simulink model "GaN_Cauer_Figure14"  (R2022b)
settings: Solver=ode15s  StartTime=-5e-6  StopTime=45e-6  MaxStep=2e-9  RelTol=1e-9  AbsTol=1e-10
model workspace (MAT data in the model file):
  C = [8e-05 0.00074 0.0065 0.002]
  R = [0.015 0.23 0.24 0.015]
settings Model: Creator=Greatlovers  LastModifiedBy=Greatlovers

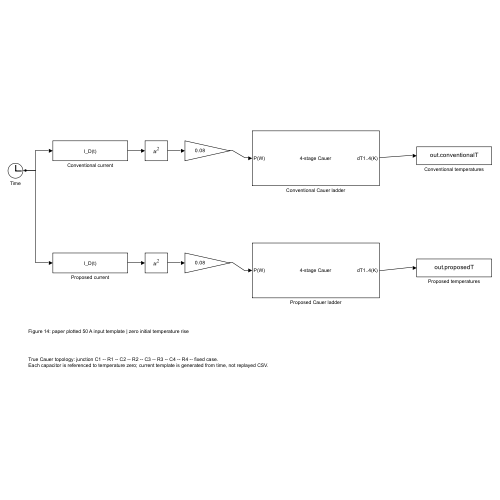
[thumbnail: Simulink's stored preview of the top-level diagram]
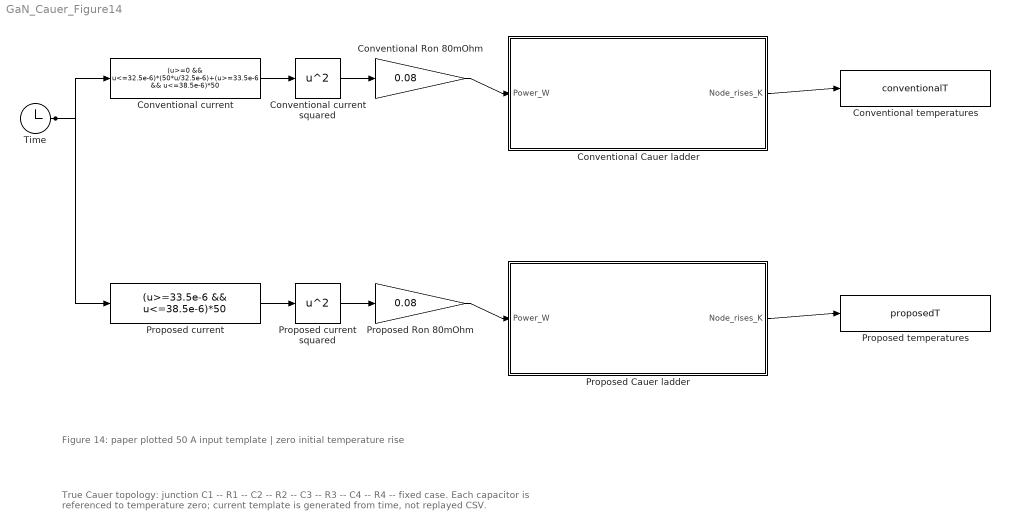
== system GaN_Cauer_Figure14 ==
  note: Figure 14: paper plotted 50 A input template | zero initial temperature rise
  note: True Cauer topology: junction C1 -- R1 -- C2 -- R2 -- C3 -- R3 -- C4 -- R4 -- fixed case.
      | Each capacitor is referenced to temperature zero; current template is generated from time, not replayed CSV.
  Conventional Cauer ladder : Subsystem
      mask Display: disp('4-stage Cauer');port_label('input',1,'P(W)');port_label('output',1,'dT1..4(K)');
  Conventional Ron 80mOhm : Gain  Gain=0.08
  Conventional current : Fcn  Expr=(u>=0 && u<=32.5e-6)*(50*u/32.5e-6)+(u>=33.5e-6 && u<=38.5e-6)*50
      mask Display: disp('I_D(t)')
  Conventional current squared : Math  Operator=square
  Conventional temperatures : ToWorkspace  VariableName=conventionalT  SaveFormat=Timeseries  SampleTime=-1
  Proposed Cauer ladder : Subsystem
      mask Display: disp('4-stage Cauer');port_label('input',1,'P(W)');port_label('output',1,'dT1..4(K)');
  Proposed Ron 80mOhm : Gain  Gain=0.08
  Proposed current : Fcn  Expr=(u>=33.5e-6 && u<=38.5e-6)*50
      mask Display: disp('I_D(t)')
  Proposed current squared : Math  Operator=square
  Proposed temperatures : ToWorkspace  VariableName=proposedT  SaveFormat=Timeseries  SampleTime=-1
  Time : Clock
  wires:
  Time/1 -> Conventional current/1, Proposed current/1
  Conventional current/1 -> Conventional current squared/1
  Conventional current squared/1 -> Conventional Ron 80mOhm/1
  Conventional Ron 80mOhm/1 -> Conventional Cauer ladder/1(Power_W)
  Conventional Cauer ladder/1(Node_rises_K) -> Conventional temperatures/1
  Proposed current/1 -> Proposed current squared/1
  Proposed current squared/1 -> Proposed Ron 80mOhm/1
  Proposed Ron 80mOhm/1 -> Proposed Cauer ladder/1(Power_W)
  Proposed Cauer ladder/1(Node_rises_K) -> Proposed temperatures/1

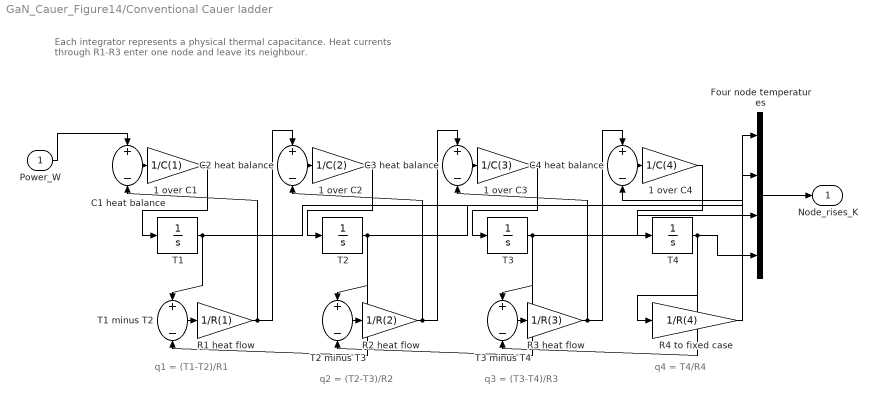
== system GaN_Cauer_Figure14/Conventional Cauer ladder ==
  note: Each integrator represents a physical thermal capacitance.
      | Heat currents through R1-R3 enter one node and leave its neighbour.
  note: q1 = (T1-T2)/R1
  note: q2 = (T2-T3)/R2
  note: q3 = (T3-T4)/R3
  note: q4 = T4/R4
  Power_W : Inport
  1 over C1 : Gain  Gain=1/C(1)
  1 over C2 : Gain  Gain=1/C(2)
  1 over C3 : Gain  Gain=1/C(3)
  1 over C4 : Gain  Gain=1/C(4)
  C1 heat balance : Sum  Inputs=+-
  C2 heat balance : Sum  Inputs=+-
  C3 heat balance : Sum  Inputs=+-
  C4 heat balance : Sum  Inputs=+-
  Four node temperatures : Mux
  R1 heat flow : Gain  Gain=1/R(1)
  R2 heat flow : Gain  Gain=1/R(2)
  R3 heat flow : Gain  Gain=1/R(3)
  R4 to fixed case : Gain  Gain=1/R(4)
  T{1..4} (4 alike) : Integrator
  T1 minus T2 : Sum  Inputs=+-
  T2 minus T3 : Sum  Inputs=+-
  T3 minus T4 : Sum  Inputs=+-
  Node_rises_K : Outport
  wires:
  C1 heat balance/1 -> 1 over C1/1
  1 over C1/1 -> T1/1
  C2 heat balance/1 -> 1 over C2/1
  1 over C2/1 -> T2/1
  C3 heat balance/1 -> 1 over C3/1
  1 over C3/1 -> T3/1
  C4 heat balance/1 -> 1 over C4/1
  1 over C4/1 -> T4/1
  Power_W/1 -> C1 heat balance/1
  T1/1 -> T1 minus T2/1, Four node temperatures/1
  T2/1 -> T1 minus T2/2, T2 minus T3/1, Four node temperatures/2
  T1 minus T2/1 -> R1 heat flow/1
  R1 heat flow/1 -> C1 heat balance/2, C2 heat balance/1
  T3/1 -> T2 minus T3/2, T3 minus T4/1, Four node temperatures/3
  T2 minus T3/1 -> R2 heat flow/1
  R2 heat flow/1 -> C2 heat balance/2, C3 heat balance/1
  T4/1 -> T3 minus T4/2, R4 to fixed case/1, Four node temperatures/4
  T3 minus T4/1 -> R3 heat flow/1
  R3 heat flow/1 -> C3 heat balance/2, C4 heat balance/1
  R4 to fixed case/1 -> C4 heat balance/2
  Four node temperatures/1 -> Node_rises_K/1

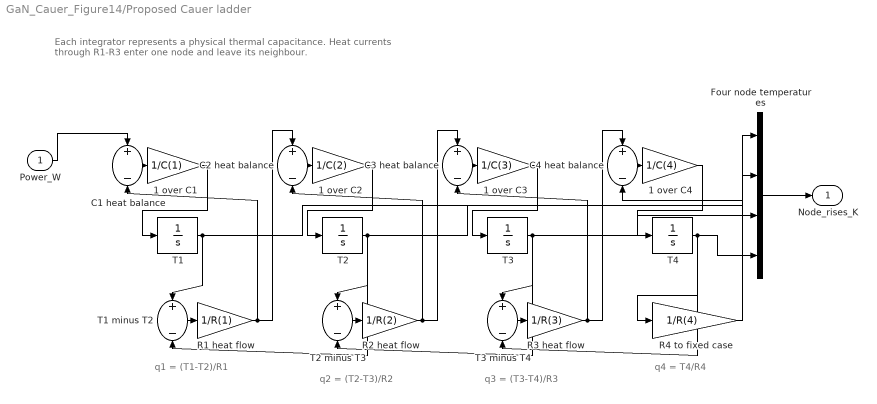
== system GaN_Cauer_Figure14/Proposed Cauer ladder ==
  note: Each integrator represents a physical thermal capacitance.
      | Heat currents through R1-R3 enter one node and leave its neighbour.
  note: q1 = (T1-T2)/R1
  note: q2 = (T2-T3)/R2
  note: q3 = (T3-T4)/R3
  note: q4 = T4/R4
  Power_W : Inport
  1 over C1 : Gain  Gain=1/C(1)
  1 over C2 : Gain  Gain=1/C(2)
  1 over C3 : Gain  Gain=1/C(3)
  1 over C4 : Gain  Gain=1/C(4)
  C1 heat balance : Sum  Inputs=+-
  C2 heat balance : Sum  Inputs=+-
  C3 heat balance : Sum  Inputs=+-
  C4 heat balance : Sum  Inputs=+-
  Four node temperatures : Mux
  R1 heat flow : Gain  Gain=1/R(1)
  R2 heat flow : Gain  Gain=1/R(2)
  R3 heat flow : Gain  Gain=1/R(3)
  R4 to fixed case : Gain  Gain=1/R(4)
  T{1..4} (4 alike) : Integrator
  T1 minus T2 : Sum  Inputs=+-
  T2 minus T3 : Sum  Inputs=+-
  T3 minus T4 : Sum  Inputs=+-
  Node_rises_K : Outport
  wires:
  C1 heat balance/1 -> 1 over C1/1
  1 over C1/1 -> T1/1
  C2 heat balance/1 -> 1 over C2/1
  1 over C2/1 -> T2/1
  C3 heat balance/1 -> 1 over C3/1
  1 over C3/1 -> T3/1
  C4 heat balance/1 -> 1 over C4/1
  1 over C4/1 -> T4/1
  Power_W/1 -> C1 heat balance/1
  T1/1 -> T1 minus T2/1, Four node temperatures/1
  T2/1 -> T1 minus T2/2, T2 minus T3/1, Four node temperatures/2
  T1 minus T2/1 -> R1 heat flow/1
  R1 heat flow/1 -> C1 heat balance/2, C2 heat balance/1
  T3/1 -> T2 minus T3/2, T3 minus T4/1, Four node temperatures/3
  T2 minus T3/1 -> R2 heat flow/1
  R2 heat flow/1 -> C2 heat balance/2, C3 heat balance/1
  T4/1 -> T3 minus T4/2, R4 to fixed case/1, Four node temperatures/4
  T3 minus T4/1 -> R3 heat flow/1
  R3 heat flow/1 -> C3 heat balance/2, C4 heat balance/1
  R4 to fixed case/1 -> C4 heat balance/2
  Four node temperatures/1 -> Node_rises_K/1
